simulink subsystem "Swerve_Drive_sub"  (R2023b)
settings: Solver=VariableStepAuto  StartTime=0.0  StopTime=10.0  RelTol=1e-3
undefined symbols (not defined in the file): Distance_BL_x, Distance_BL_y, Distance_BR_x, Distance_BR_y, Distance_FL_x, Distance_FL_y, Distance_FR_x, Distance_FR_y, Drive_Wheel_Max_Speed, Steering_Heading_Control_Deadzone
libraries: Controls_Components_lib x9, simulink x1
settings Model: Creator=ander  LastModifiedBy=ander

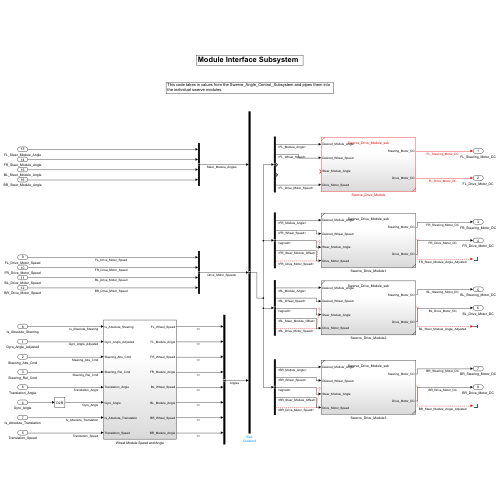
[thumbnail: Simulink's stored preview of the top-level diagram]
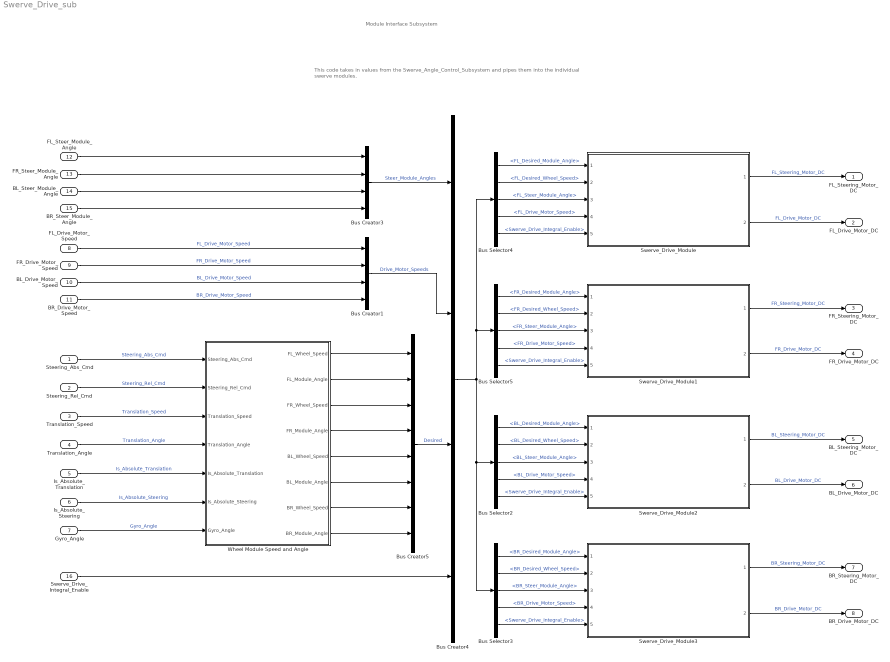
== system Swerve_Drive_sub ==
  note: This code takes in values from the Swerve_Angle_Control_Subsystem and pipes them into the individual swerve modules.
  note: Module Interface Subsystem
  Steering_Abs_Cmd : Inport
  Steering_Rel_Cmd : Inport  Port=2
  Translation_Speed : Inport  Port=3
  Translation_Angle : Inport  Port=4
  Is_Absolute_Translation : Inport  Port=5
  Is_Absolute_Steering : Inport  Port=6
  Gyro_Angle : Inport  Port=7
  FL_Drive_Motor_Speed : Inport  Port=8
  FR_Drive_Motor_Speed : Inport  Port=9
  BL_Drive_Motor_Speed : Inport  Port=10
  BR_Drive_Motor_Speed : Inport  Port=11
  FL_Steer_Module_Angle : Inport  Port=12
  FR_Steer_Module_Angle : Inport  Port=13
  BL_Steer_Module_Angle : Inport  Port=14
  BR_Steer_Module_Angle : Inport  Port=15
  Swerve_Drive_Integral_Enable : Inport  Port=16
  Bus Creator1 : BusCreator  Inputs=4
  Bus Creator3 : BusCreator  Inputs=4
  Bus Creator4 : BusCreator  Inputs=4
  Bus Creator5 : BusCreator  Inputs=8
  Bus Selector2 : BusSelector  OutputSignals=Desired.BL_Desired_Module_Angle,Desired.BL_Desired_Wheel_Speed,Steer_Module_Angles.BL_Steer_Module_Angle,Drive_Motor_Speeds.BL_Drive_Motor_Speed,Swerve_Drive_Integral_Enable
  Bus Selector3 : BusSelector  OutputSignals=Desired.BR_Desired_Module_Angle,Desired.BR_Desired_Wheel_Speed,Steer_Module_Angles.BR_Steer_Module_Angle,Drive_Motor_Speeds.BR_Drive_Motor_Speed,Swerve_Drive_Integral_Enable
  Bus Selector4 : BusSelector  OutputSignals=Desired.FL_Desired_Module_Angle,Desired.FL_Desired_Wheel_Speed,Steer_Module_Angles.FL_Steer_Module_Angle,Drive_Motor_Speeds.FL_Drive_Motor_Speed,Swerve_Drive_Integral_Enable
  Bus Selector5 : BusSelector  OutputSignals=Desired.FR_Desired_Module_Angle,Desired.FR_Desired_Wheel_Speed,Steer_Module_Angles.FR_Steer_Module_Angle,Drive_Motor_Speeds.FR_Drive_Motor_Speed,Swerve_Drive_Integral_Enable
  Swerve_Drive_Module{,1..3} (4 alike) : Subsystem  ReferencedSubsystem=Swerve_Drive_Module_sub
  Wheel Module Speed and Angle : Subsystem
  FL_Steering_Motor_DC : Outport
  FL_Drive_Motor_DC : Outport  Port=2
  FR_Steering_Motor_DC : Outport  Port=3
  FR_Drive_Motor_DC : Outport  Port=4
  BL_Steering_Motor_DC : Outport  Port=5
  BL_Drive_Motor_DC : Outport  Port=6
  BR_Steering_Motor_DC : Outport  Port=7
  BR_Drive_Motor_DC : Outport  Port=8
  wires:
  Swerve_Drive_Module/1 -> FL_Steering_Motor_DC/1  "FL_Steering_Motor_DC"
  Swerve_Drive_Module2/2 -> BL_Drive_Motor_DC/1  "BL_Drive_Motor_DC"
  Swerve_Drive_Module1/1 -> FR_Steering_Motor_DC/1  "FR_Steering_Motor_DC"
  Swerve_Drive_Module3/2 -> BR_Drive_Motor_DC/1  "BR_Drive_Motor_DC"
  Swerve_Drive_Module3/1 -> BR_Steering_Motor_DC/1  "BR_Steering_Motor_DC"
  Swerve_Drive_Module1/2 -> FR_Drive_Motor_DC/1  "FR_Drive_Motor_DC"
  Swerve_Drive_Module2/1 -> BL_Steering_Motor_DC/1  "BL_Steering_Motor_DC"
  Swerve_Drive_Module/2 -> FL_Drive_Motor_DC/1  "FL_Drive_Motor_DC"
  Bus Selector3/2 -> Swerve_Drive_Module3/2  "<BR_Desired_Wheel_Speed>"
  Bus Selector3/1 -> Swerve_Drive_Module3/1  "<BR_Desired_Module_Angle>"
  Bus Selector2/2 -> Swerve_Drive_Module2/2  "<BL_Desired_Wheel_Speed>"
  Bus Selector2/1 -> Swerve_Drive_Module2/1  "<BL_Desired_Module_Angle>"
  Bus Selector5/2 -> Swerve_Drive_Module1/2  "<FR_Desired_Wheel_Speed>"
  Bus Selector5/1 -> Swerve_Drive_Module1/1  "<FR_Desired_Module_Angle>"
  Bus Selector4/4 -> Swerve_Drive_Module/4  "<FL_Drive_Motor_Speed>"
  Bus Selector4/2 -> Swerve_Drive_Module/2  "<FL_Desired_Wheel_Speed>"
  Bus Selector4/1 -> Swerve_Drive_Module/1  "<FL_Desired_Module_Angle>"
  Bus Creator4/1 -> Bus Selector5/1, Bus Selector4/1, Bus Selector2/1, Bus Selector3/1
  Bus Creator3/1 -> Bus Creator4/1  "Steer_Module_Angles"
  Bus Creator1/1 -> Bus Creator4/2  "Drive_Motor_Speeds"
  Bus Creator5/1 -> Bus Creator4/3  "Desired"
  BR_Steer_Module_Angle/1 -> Bus Creator3/4
  BL_Steer_Module_Angle/1 -> Bus Creator3/3
  FR_Steer_Module_Angle/1 -> Bus Creator3/2
  FL_Steer_Module_Angle/1 -> Bus Creator3/1
  FL_Drive_Motor_Speed/1 -> Bus Creator1/1  "FL_Drive_Motor_Speed"
  FR_Drive_Motor_Speed/1 -> Bus Creator1/2  "FR_Drive_Motor_Speed"
  BL_Drive_Motor_Speed/1 -> Bus Creator1/3  "BL_Drive_Motor_Speed"
  BR_Drive_Motor_Speed/1 -> Bus Creator1/4  "BR_Drive_Motor_Speed"
  Is_Absolute_Steering/1 -> Wheel Module Speed and Angle/6(Is_Absolute_Steering)  "Is_Absolute_Steering"
  Steering_Abs_Cmd/1 -> Wheel Module Speed and Angle/1(Steering_Abs_Cmd)  "Steering_Abs_Cmd"
  Steering_Rel_Cmd/1 -> Wheel Module Speed and Angle/2(Steering_Rel_Cmd)  "Steering_Rel_Cmd"
  Translation_Angle/1 -> Wheel Module Speed and Angle/4(Translation_Angle)  "Translation_Angle"
  Is_Absolute_Translation/1 -> Wheel Module Speed and Angle/5(Is_Absolute_Translation)  "Is_Absolute_Translation"
  Translation_Speed/1 -> Wheel Module Speed and Angle/3(Translation_Speed)  "Translation_Speed"
  Wheel Module Speed and Angle/1(FL_Wheel_Speed) -> Bus Creator5/1
  Wheel Module Speed and Angle/2(FL_Module_Angle) -> Bus Creator5/2
  Wheel Module Speed and Angle/3(FR_Wheel_Speed) -> Bus Creator5/3
  Wheel Module Speed and Angle/4(FR_Module_Angle) -> Bus Creator5/4
  Wheel Module Speed and Angle/5(BL_Wheel_Speed) -> Bus Creator5/5
  Wheel Module Speed and Angle/6(BL_Module_Angle) -> Bus Creator5/6
  Wheel Module Speed and Angle/7(BR_Wheel_Speed) -> Bus Creator5/7
  Wheel Module Speed and Angle/8(BR_Module_Angle) -> Bus Creator5/8
  Gyro_Angle/1 -> Wheel Module Speed and Angle/7(Gyro_Angle)  "Gyro_Angle"
  Bus Selector4/3 -> Swerve_Drive_Module/3  "<FL_Steer_Module_Angle>"
  Bus Selector5/3 -> Swerve_Drive_Module1/3  "<FR_Steer_Module_Angle>"
  Bus Selector5/4 -> Swerve_Drive_Module1/4  "<FR_Drive_Motor_Speed>"
  Bus Selector2/3 -> Swerve_Drive_Module2/3  "<BL_Steer_Module_Angle>"
  Bus Selector2/4 -> Swerve_Drive_Module2/4  "<BL_Drive_Motor_Speed>"
  Bus Selector3/3 -> Swerve_Drive_Module3/3  "<BR_Steer_Module_Angle>"
  Bus Selector3/4 -> Swerve_Drive_Module3/4  "<BR_Drive_Motor_Speed>"
  Swerve_Drive_Integral_Enable/1 -> Bus Creator4/4
  Bus Selector4/5 -> Swerve_Drive_Module/5  "<Swerve_Drive_Integral_Enable>"
  Bus Selector5/5 -> Swerve_Drive_Module1/5  "<Swerve_Drive_Integral_Enable>"
  Bus Selector2/5 -> Swerve_Drive_Module2/5  "<Swerve_Drive_Integral_Enable>"
  Bus Selector3/5 -> Swerve_Drive_Module3/5  "<Swerve_Drive_Integral_Enable>"

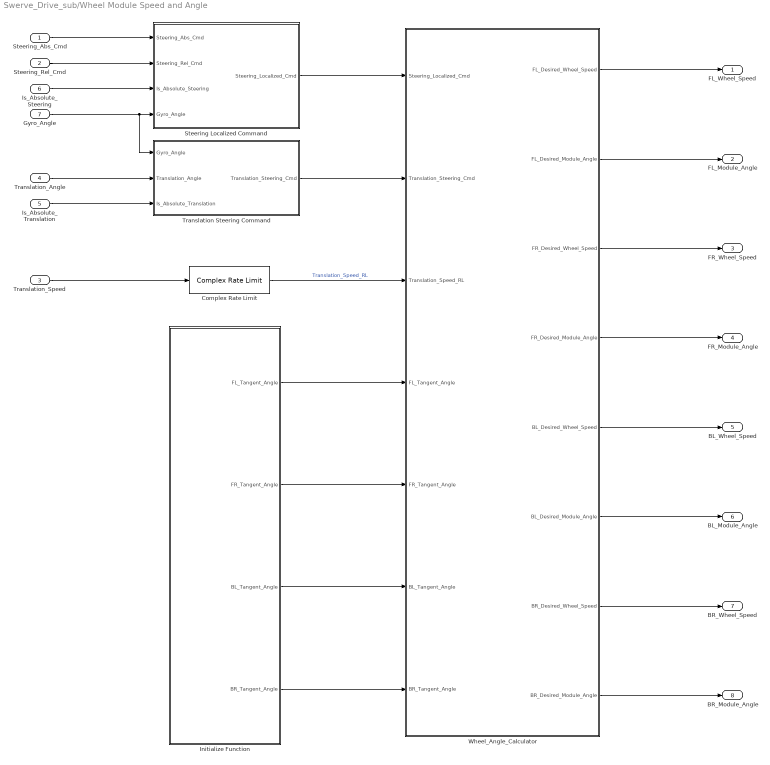
== system Swerve_Drive_sub/Wheel Module Speed and Angle ==
  Steering_Abs_Cmd : Inport
  Steering_Rel_Cmd : Inport  Port=2
  Translation_Speed : Inport  Port=3
  Translation_Angle : Inport  Port=4
  Is_Absolute_Translation : Inport  Port=5
  Is_Absolute_Steering : Inport  Port=6
  Gyro_Angle : Inport  Port=7
  Complex Rate Limit : Controls_Components_lib/Complex Rate Limit  Rate_Limit_Inc=Translation_Speed_Rate_Limit_Inc  Rate_Limit_Dec=Translation_Speed_Rate_Limit_Dec  Approaching_Zero_Error_Threshold=Translation_Speed_Approach_Zero_Error_Thresh  Approaching_Zero_Final_Scale_Factor=Translation_Speed_Approach_Zero_Final_Thresh  Approaching_NonZero_Error_Threshold=Translation_Speed_NonZero_Error_Thresh  Approaching_NonZero_Final_Scale_Factor=Translation_Speed_NonZero_Final_Scale_Factor
  Initialize Function : Subsystem  TreatAsAtomicUnit=on
  Steering Localized Command : Subsystem
  Translation Steering Command : Subsystem
  Wheel_Angle_Calculator : Subsystem
  FL_Wheel_Speed : Outport
  FL_Module_Angle : Outport  Port=2
  FR_Wheel_Speed : Outport  Port=3
  FR_Module_Angle : Outport  Port=4
  BL_Wheel_Speed : Outport  Port=5
  BL_Module_Angle : Outport  Port=6
  BR_Wheel_Speed : Outport  Port=7
  BR_Module_Angle : Outport  Port=8
  wires:
  Complex Rate Limit/1 -> Wheel_Angle_Calculator/3(Translation_Speed_RL)  "Translation_Speed_RL"
  Translation_Speed/1 -> Complex Rate Limit/1
  Is_Absolute_Steering/1 -> Steering Localized Command/3(Is_Absolute_Steering)
  Steering_Rel_Cmd/1 -> Steering Localized Command/2(Steering_Rel_Cmd)
  Wheel_Angle_Calculator/2(FL_Desired_Module_Angle) -> FL_Module_Angle/1
  Wheel_Angle_Calculator/4(FR_Desired_Module_Angle) -> FR_Module_Angle/1
  Wheel_Angle_Calculator/6(BL_Desired_Module_Angle) -> BL_Module_Angle/1
  Steering Localized Command/1(Steering_Localized_Cmd) -> Wheel_Angle_Calculator/1(Steering_Localized_Cmd)
  Wheel_Angle_Calculator/3(FR_Desired_Wheel_Speed) -> FR_Wheel_Speed/1
  Wheel_Angle_Calculator/1(FL_Desired_Wheel_Speed) -> FL_Wheel_Speed/1
  Wheel_Angle_Calculator/7(BR_Desired_Wheel_Speed) -> BR_Wheel_Speed/1
  Is_Absolute_Translation/1 -> Translation Steering Command/3(Is_Absolute_Translation)
  Initialize Function/4(BR_Tangent_Angle) -> Wheel_Angle_Calculator/7(BR_Tangent_Angle)
  Initialize Function/2(FR_Tangent_Angle) -> Wheel_Angle_Calculator/5(FR_Tangent_Angle)
  Wheel_Angle_Calculator/8(BR_Desired_Module_Angle) -> BR_Module_Angle/1
  Initialize Function/3(BL_Tangent_Angle) -> Wheel_Angle_Calculator/6(BL_Tangent_Angle)
  Steering_Abs_Cmd/1 -> Steering Localized Command/1(Steering_Abs_Cmd)
  Wheel_Angle_Calculator/5(BL_Desired_Wheel_Speed) -> BL_Wheel_Speed/1
  Gyro_Angle/1 -> Steering Localized Command/4(Gyro_Angle), Translation Steering Command/1(Gyro_Angle)
  Initialize Function/1(FL_Tangent_Angle) -> Wheel_Angle_Calculator/4(FL_Tangent_Angle)
  Translation Steering Command/1(Translation_Steering_Cmd) -> Wheel_Angle_Calculator/2(Translation_Steering_Cmd)
  Translation_Angle/1 -> Translation Steering Command/2(Translation_Angle)

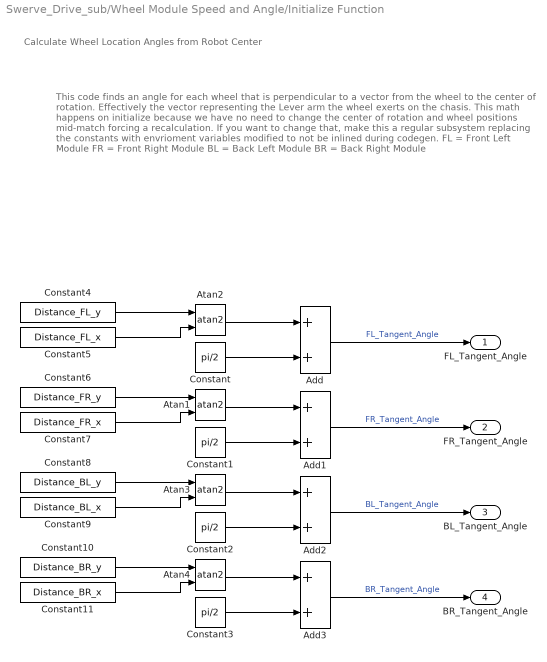
== system Swerve_Drive_sub/Wheel Module Speed and Angle/Initialize Function ==
  note: This code finds an angle for each wheel that is perpendicular to a vector from the wheel to the center of rotation. Effectively the vector representing the Lever arm the wheel exerts on the chasis. This math happens on initialize because we have no need to change the center of rotation and wheel positions mid-match forcing a recalculation. If you want to change that, make this a regular subsystem replacing the constants with envrioment variables modified to not be inlined during codegen.
      | FL = Front Left Module
      | FR = Front Right Module
      | BL = Back Left Module
      | BR = Back Right Module
  note: Calculate Wheel Location Angles from Robot Center
  Add{,1..3} (4 alike) : Sum
  Atan{1..4} (4 alike) : Trigonometry  Operator=atan2
  Constant{,1..3} (4 alike) : Constant  Value=pi/2
  Constant10 : Constant  Value=Distance_BR_y
  Constant11 : Constant  Value=Distance_BR_x
  Constant4 : Constant  Value=Distance_FL_y
  Constant5 : Constant  Value=Distance_FL_x
  Constant6 : Constant  Value=Distance_FR_y
  Constant7 : Constant  Value=Distance_FR_x
  Constant8 : Constant  Value=Distance_BL_y
  Constant9 : Constant  Value=Distance_BL_x
  FL_Tangent_Angle : Outport
  FR_Tangent_Angle : Outport  Port=2
  BL_Tangent_Angle : Outport  Port=3
  BR_Tangent_Angle : Outport  Port=4
  wires:
  Constant11/1 -> Atan4/2
  Constant10/1 -> Atan4/1
  Constant9/1 -> Atan3/2
  Constant8/1 -> Atan3/1
  Constant7/1 -> Atan1/2
  Constant6/1 -> Atan1/1
  Constant5/1 -> Atan2/2
  Constant4/1 -> Atan2/1
  Atan4/1 -> Add3/1
  Constant3/1 -> Add3/2
  Constant2/1 -> Add2/2
  Atan3/1 -> Add2/1
  Atan1/1 -> Add1/1
  Constant1/1 -> Add1/2
  Constant/1 -> Add/2
  Atan2/1 -> Add/1
  Add/1 -> FL_Tangent_Angle/1  "FL_Tangent_Angle"
  Add1/1 -> FR_Tangent_Angle/1  "FR_Tangent_Angle"
  Add2/1 -> BL_Tangent_Angle/1  "BL_Tangent_Angle"
  Add3/1 -> BR_Tangent_Angle/1  "BR_Tangent_Angle"

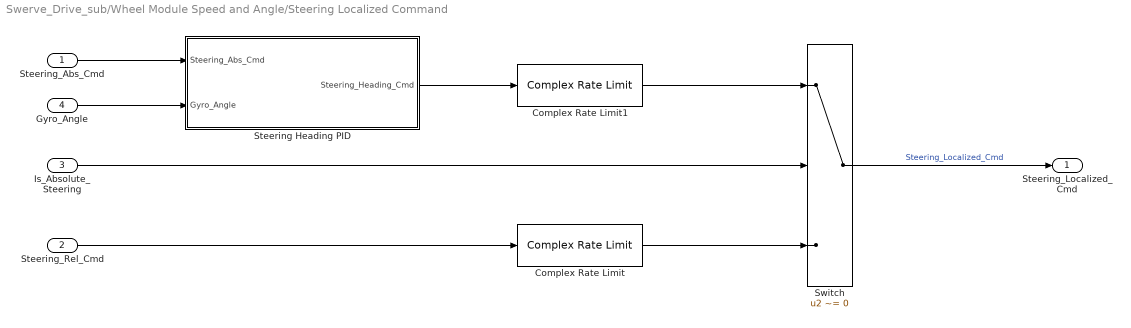
== system Swerve_Drive_sub/Wheel Module Speed and Angle/Steering Localized Command ==
  Steering_Abs_Cmd : Inport
  Steering_Rel_Cmd : Inport  Port=2
  Is_Absolute_Steering : Inport  Port=3
  Gyro_Angle : Inport  Port=4
  Complex Rate Limit : Controls_Components_lib/Complex Rate Limit  Rate_Limit_Inc=Steering_Relative_Cmd_Rate_Limit_Inc  Rate_Limit_Dec=Steering_Relative_Cmd_Rate_Limit_Dec  Approaching_Zero_Error_Threshold=Steering_Relative_Cmd_Approach_Zero_Error_Thresh  Approaching_Zero_Final_Scale_Factor=Steering_Relative_Cmd_Approach_Zero_Final_Thresh  Approaching_NonZero_Error_Threshold=Steering_Relative_Cmd_NonZero_Error_Thresh  Approaching_NonZero_Final_Scale_Factor=Steering_Relative_Cmd_NonZero_Final_Scale_Factor
  Complex Rate Limit1 : Controls_Components_lib/Complex Rate Limit  Rate_Limit_Inc=Steering_Absolute_Cmd_Rate_Limit_Inc  Rate_Limit_Dec=Steering_Absolute_Cmd_Rate_Limit_Dec  Approaching_Zero_Error_Threshold=Steering_Absolute_Cmd_Approach_Zero_Error_Thresh  Approaching_Zero_Final_Scale_Factor=Steering_Absolute_Cmd_Approach_Zero_Final_Thresh  Approaching_NonZero_Error_Threshold=Steering_Absolute_Cmd_NonZero_Error_Thresh  Approaching_NonZero_Final_Scale_Factor=Steering_Absolute_Cmd_NonZero_Final_Scale_Factor
  Steering Heading PID : Subsystem
  Switch : Switch  Criteria=u2 ~= 0  SaturateOnIntegerOverflow=off  InputSameDT=off
  Steering_Localized_Cmd : Outport
  wires:
  Complex Rate Limit1/1 -> Switch/1
  Complex Rate Limit/1 -> Switch/3
  Gyro_Angle/1 -> Steering Heading PID/2(Gyro_Angle)
  Switch/1 -> Steering_Localized_Cmd/1  "Steering_Localized_Cmd"
  Steering_Rel_Cmd/1 -> Complex Rate Limit/1
  Steering Heading PID/1(Steering_Heading_Cmd) -> Complex Rate Limit1/1
  Is_Absolute_Steering/1 -> Switch/2
  Steering_Abs_Cmd/1 -> Steering Heading PID/1(Steering_Abs_Cmd)

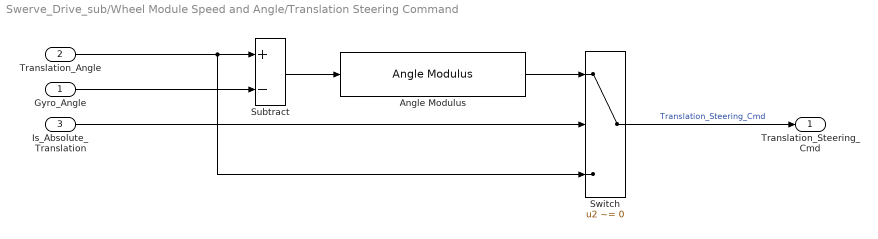
== system Swerve_Drive_sub/Wheel Module Speed and Angle/Translation Steering Command ==
  Gyro_Angle : Inport
  Translation_Angle : Inport  Port=2
  Is_Absolute_Translation : Inport  Port=3
  Angle Modulus : Controls_Components_lib/Angle Modulus  SystemSampleTime=-1  VariantActivationTime=update diagram  AllowFlexibleInterface=on  Latency=0  AutoFrameSizeCalculation=off
  Subtract : Sum  Inputs=+-
  Switch : Switch  Criteria=u2 ~= 0  SaturateOnIntegerOverflow=off  InputSameDT=off
  Translation_Steering_Cmd : Outport
  wires:
  Subtract/1 -> Angle Modulus/1
  Translation_Angle/1 -> Switch/3, Subtract/1
  Angle Modulus/1 -> Switch/1
  Switch/1 -> Translation_Steering_Cmd/1  "Translation_Steering_Cmd"
  Gyro_Angle/1 -> Subtract/2
  Is_Absolute_Translation/1 -> Switch/2

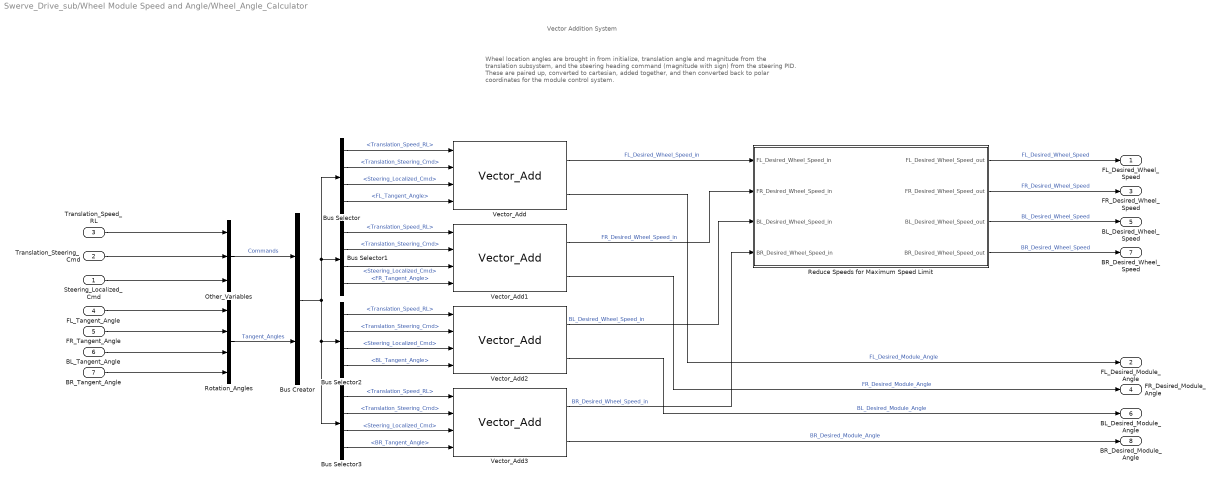
== system Swerve_Drive_sub/Wheel Module Speed and Angle/Wheel_Angle_Calculator ==
  note: Wheel location angles are brought in from initialize, translation angle and magnitude from the translation subsystem, and the steering heading command (magnitude with sign) from the steering PID. These are paired up, converted to cartesian, added together, and then converted back to polar coordinates for the module control system.
  note: Vector Addition System
  Steering_Localized_Cmd : Inport
  Translation_Steering_Cmd : Inport  Port=2
  Translation_Speed_RL : Inport  Port=3
  FL_Tangent_Angle : Inport  Port=4
  FR_Tangent_Angle : Inport  Port=5
  BL_Tangent_Angle : Inport  Port=6
  BR_Tangent_Angle : Inport  Port=7
  Bus Creator : BusCreator  Inputs=2
  Bus Selector : BusSelector  OutputSignals=Commands.Translation_Speed_RL,Commands.Translation_Steering_Cmd,Commands.Steering_Localized_Cmd,Tangent_Angles.FL_Tangent_Angle
  Bus Selector1 : BusSelector  OutputSignals=Commands.Translation_Speed_RL,Commands.Translation_Steering_Cmd,Commands.Steering_Localized_Cmd,Tangent_Angles.FR_Tangent_Angle
  Bus Selector2 : BusSelector  OutputSignals=Commands.Translation_Speed_RL,Commands.Translation_Steering_Cmd,Commands.Steering_Localized_Cmd,Tangent_Angles.BL_Tangent_Angle
  Bus Selector3 : BusSelector  OutputSignals=Commands.Translation_Speed_RL,Commands.Translation_Steering_Cmd,Commands.Steering_Localized_Cmd,Tangent_Angles.BR_Tangent_Angle
  Other_Variables : BusCreator  Inputs=3
  Reduce Speeds for Maximum Speed Limit : Subsystem
  Rotation_Angles : BusCreator  Inputs=4
  Vector_Add{,1..3} (4 alike) : Controls_Components_lib/Vector_Add  SystemSampleTime=-1  VariantActivationTime=update diagram  AllowFlexibleInterface=on  Latency=0  AutoFrameSizeCalculation=off
  FL_Desired_Wheel_Speed : Outport
  FL_Desired_Module_Angle : Outport  Port=2
  FR_Desired_Wheel_Speed : Outport  Port=3
  FR_Desired_Module_Angle : Outport  Port=4
  BL_Desired_Wheel_Speed : Outport  Port=5
  BL_Desired_Module_Angle : Outport  Port=6
  BR_Desired_Wheel_Speed : Outport  Port=7
  BR_Desired_Module_Angle : Outport  Port=8
  wires:
  Vector_Add3/1 -> Reduce Speeds for Maximum Speed Limit/4(BR_Desired_Wheel_Speed_in)  "BR_Desired_Wheel_Speed_in"
  Vector_Add2/1 -> Reduce Speeds for Maximum Speed Limit/3(BL_Desired_Wheel_Speed_in)  "BL_Desired_Wheel_Speed_in"
  Vector_Add1/1 -> Reduce Speeds for Maximum Speed Limit/2(FR_Desired_Wheel_Speed_in)  "FR_Desired_Wheel_Speed_in"
  Vector_Add/1 -> Reduce Speeds for Maximum Speed Limit/1(FL_Desired_Wheel_Speed_in)  "FL_Desired_Wheel_Speed_in"
  Reduce Speeds for Maximum Speed Limit/4(BR_Desired_Wheel_Speed_out) -> BR_Desired_Wheel_Speed/1  "BR_Desired_Wheel_Speed"
  Reduce Speeds for Maximum Speed Limit/3(BL_Desired_Wheel_Speed_out) -> BL_Desired_Wheel_Speed/1  "BL_Desired_Wheel_Speed"
  Reduce Speeds for Maximum Speed Limit/2(FR_Desired_Wheel_Speed_out) -> FR_Desired_Wheel_Speed/1  "FR_Desired_Wheel_Speed"
  Reduce Speeds for Maximum Speed Limit/1(FL_Desired_Wheel_Speed_out) -> FL_Desired_Wheel_Speed/1  "FL_Desired_Wheel_Speed"
  Steering_Localized_Cmd/1 -> Other_Variables/3
  Translation_Steering_Cmd/1 -> Other_Variables/2
  Translation_Speed_RL/1 -> Other_Variables/1
  FR_Tangent_Angle/1 -> Rotation_Angles/2
  FL_Tangent_Angle/1 -> Rotation_Angles/1
  BL_Tangent_Angle/1 -> Rotation_Angles/3
  BR_Tangent_Angle/1 -> Rotation_Angles/4
  Other_Variables/1 -> Bus Creator/1  "Commands"
  Rotation_Angles/1 -> Bus Creator/2  "Tangent_Angles"
  Bus Creator/1 -> Bus Selector/1, Bus Selector1/1, Bus Selector3/1, Bus Selector2/1
  Bus Selector/2 -> Vector_Add/2  "<Translation_Steering_Cmd>"
  Bus Selector/1 -> Vector_Add/1  "<Translation_Speed_RL>"
  Bus Selector/3 -> Vector_Add/3  "<Steering_Localized_Cmd>"
  Bus Selector/4 -> Vector_Add/4  "<FL_Tangent_Angle>"
  Bus Selector1/1 -> Vector_Add1/1  "<Translation_Speed_RL>"
  Bus Selector1/2 -> Vector_Add1/2  "<Translation_Steering_Cmd>"
  Bus Selector1/3 -> Vector_Add1/3  "<Steering_Localized_Cmd>"
  Bus Selector1/4 -> Vector_Add1/4  "<FR_Tangent_Angle>"
  Bus Selector2/1 -> Vector_Add2/1  "<Translation_Speed_RL>"
  Bus Selector2/2 -> Vector_Add2/2  "<Translation_Steering_Cmd>"
  Bus Selector2/3 -> Vector_Add2/3  "<Steering_Localized_Cmd>"
  Bus Selector2/4 -> Vector_Add2/4  "<BL_Tangent_Angle>"
  Bus Selector3/1 -> Vector_Add3/1  "<Translation_Speed_RL>"
  Bus Selector3/2 -> Vector_Add3/2  "<Translation_Steering_Cmd>"
  Bus Selector3/3 -> Vector_Add3/3  "<Steering_Localized_Cmd>"
  Bus Selector3/4 -> Vector_Add3/4  "<BR_Tangent_Angle>"
  Vector_Add/2 -> FL_Desired_Module_Angle/1  "FL_Desired_Module_Angle"
  Vector_Add1/2 -> FR_Desired_Module_Angle/1  "FR_Desired_Module_Angle"
  Vector_Add2/2 -> BL_Desired_Module_Angle/1  "BL_Desired_Module_Angle"
  Vector_Add3/2 -> BR_Desired_Module_Angle/1  "BR_Desired_Module_Angle"

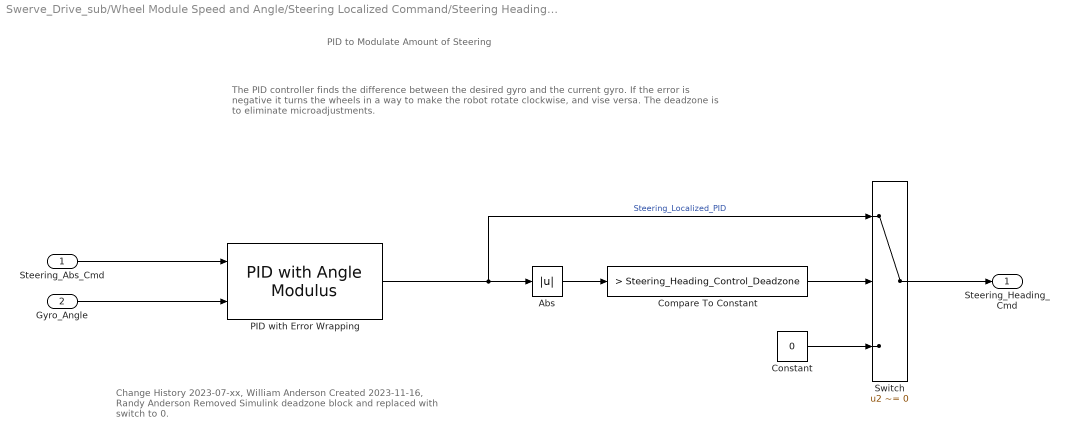
== system Swerve_Drive_sub/Wheel Module Speed and Angle/Steering Localized Command/Steering Heading PID ==
  note: PID to Modulate Amount of Steering
  note: The PID controller finds the difference between the desired gyro and the current gyro. If the error is negative it turns the wheels in a way to make the robot rotate clockwise, and vise versa.
      |
      | The deadzone is to eliminate microadjustments.
  note: Change History
      | 2023-07-xx, William Anderson
      | Created
      | 2023-11-16, Randy Anderson
      | Removed Simulink deadzone block and replaced with switch to 0.
  Steering_Abs_Cmd : Inport
  Gyro_Angle : Inport  Port=2
  Abs : Abs  SaturateOnIntegerOverflow=off
  Compare To Constant : simulink/Logic and Bit Operations/Compare To Constant  relop=>  const=Steering_Heading_Control_Deadzone  OutDataTypeStr=boolean
  Constant : Constant  Value=0
  PID with Error Wrapping : Controls_Components_lib/PID with Angle Modulus  Gain_P=Steering_Heading_Control_P  Gain_I=Steering_Heading_Control_I  Gain_D=Steering_Heading_Control_D  FilterCoeff_D=Steering_Heading_Control_D_FilterCoeff  Limit_I_Upper=Steering_Heading_Control_I_UL  Limit_I_Lower=Steering_Heading_Control_I_LL  Limit_D_Upper=Steering_Heading_Control_D_UL  Limit_D_Lower=Steering_Heading_Control_D_LL  Limit_T_Upper=Steering_Heading_Control_Total_UL  Limit_T_Lower=Steering_Heading_Control_Total_LL
  Switch : Switch  Criteria=u2 ~= 0  SaturateOnIntegerOverflow=off  InputSameDT=off
  Steering_Heading_Cmd : Outport
  wires:
  Abs/1 -> Compare To Constant/1
  Compare To Constant/1 -> Switch/2
  Switch/1 -> Steering_Heading_Cmd/1
  Constant/1 -> Switch/3
  PID with Error Wrapping/1 -> Abs/1, Switch/1  "Steering_Localized_PID"
  Steering_Abs_Cmd/1 -> PID with Error Wrapping/1
  Gyro_Angle/1 -> PID with Error Wrapping/2

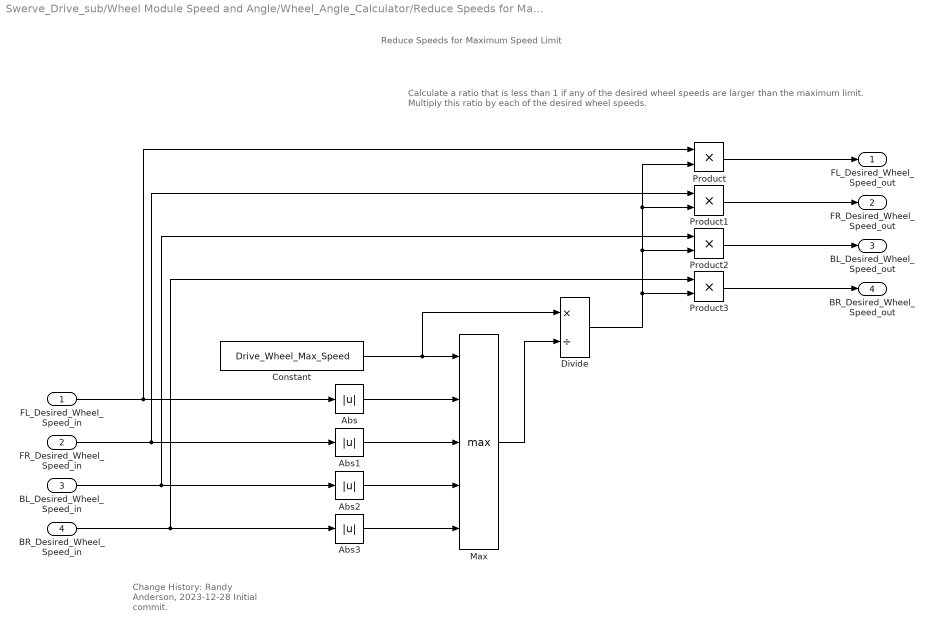
== system Swerve_Drive_sub/Wheel Module Speed and Angle/Wheel_Angle_Calculator/Reduce Speeds for Maximum Speed Limit ==
  note: Reduce Speeds for Maximum Speed Limit
  note: Calculate a ratio that is less than 1 if any of the desired wheel speeds are larger than the maximum limit. Multiply this ratio by each of the desired wheel speeds.
  note: Change History:
      | Randy Anderson, 2023-12-28
      |     Initial commit.
  FL_Desired_Wheel_Speed_in : Inport
  FR_Desired_Wheel_Speed_in : Inport  Port=2
  BL_Desired_Wheel_Speed_in : Inport  Port=3
  BR_Desired_Wheel_Speed_in : Inport  Port=4
  Abs{,1..3} (4 alike) : Abs  SaturateOnIntegerOverflow=off
  Constant : Constant  Value=Drive_Wheel_Max_Speed
  Divide : Product  Inputs=*/
  Max : MinMax  Function=max  Inputs=5
  Product{,1..3} (4 alike) : Product
  FL_Desired_Wheel_Speed_out : Outport
  FR_Desired_Wheel_Speed_out : Outport  Port=2
  BL_Desired_Wheel_Speed_out : Outport  Port=3
  BR_Desired_Wheel_Speed_out : Outport  Port=4
  wires:
  Product3/1 -> BR_Desired_Wheel_Speed_out/1
  Product2/1 -> BL_Desired_Wheel_Speed_out/1
  Product1/1 -> FR_Desired_Wheel_Speed_out/1
  Product/1 -> FL_Desired_Wheel_Speed_out/1
  Divide/1 -> Product3/2, Product2/2, Product1/2, Product/2
  Constant/1 -> Max/1, Divide/1
  Max/1 -> Divide/2
  Abs3/1 -> Max/5
  Abs2/1 -> Max/4
  Abs/1 -> Max/2
  Abs1/1 -> Max/3
  BR_Desired_Wheel_Speed_in/1 -> Abs3/1, Product3/1
  BL_Desired_Wheel_Speed_in/1 -> Abs2/1, Product2/1
  FR_Desired_Wheel_Speed_in/1 -> Abs1/1, Product1/1
  FL_Desired_Wheel_Speed_in/1 -> Product/1, Abs/1
